simulink model "HEMS_1GDL_DISCRETIZADO"  (R2026b)
settings: Solver=VariableStepAuto  StopTime=5  MaxStep=1e-4
undefined symbols (not defined in the file): airgap_bp, airgap_zero_current, current_bp, Fz_table, g0, I_ff, I_initial, I_max, Kd_cur, Kd_pos, Ki_cur, Ki_pos, Kp_cur, Kp_pos, L_coil, m, N_pos, R_coil, Ts_cur, Ts_pos, v_initial, V_max, z_initial
libraries: slpidlib x2
settings Model: Creator=34666  LastModifiedBy=34666

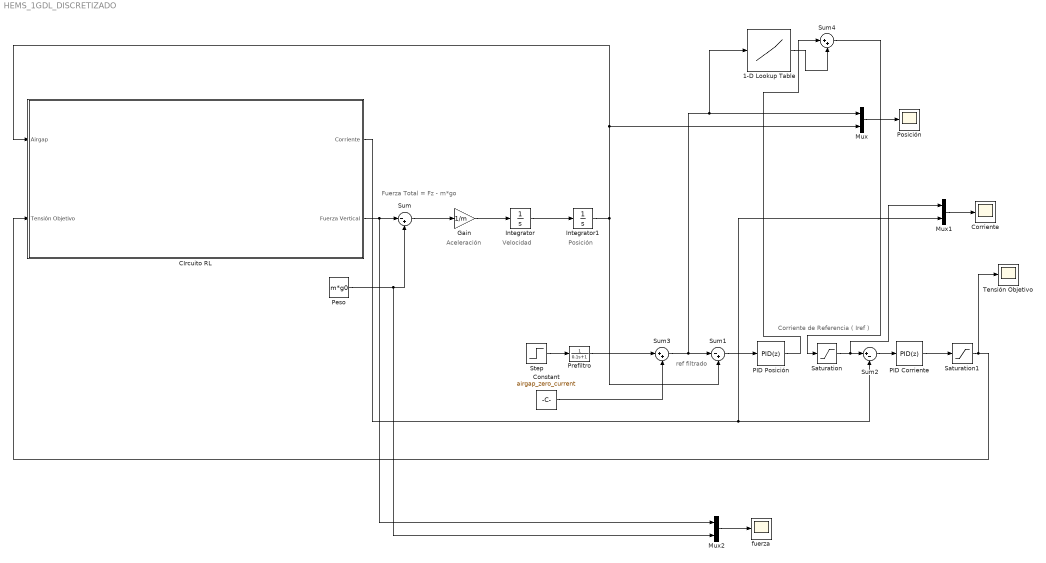
== system HEMS_1GDL_DISCRETIZADO ==
  note: ref filtrado
  note: Corriente de Referencia ( Iref )
  note: Aceleración
  note: Fuerza Total = Fz - m*go
  note: Velocidad
  note: Posición
  1-D Lookup Table : Lookup_n-D  NumberOfTableDimensions=1  BreakpointsForDimension1=airgap_bp  Table=I_ff  ExtrapMethod=Clip  InternalRulePriority=Speed  RndMeth=Simplest
  CIrcuito RL : Subsystem
  Constant : Constant  Value=airgap_zero_current
  Corriente : Scope
      settings: ActiveDisplayYMinimum=-30.569144829909195  ActiveDisplayYMaximum=22.357809311337615  DataLoggingVariableName=ScopeData2
  Gain : Gain  Gain=1/m
  Integrator : Integrator  InitialCondition=v_initial
  Integrator1 : Integrator  InitialCondition=z_initial
  Mux : Mux  Inputs=2
  Mux1 : Mux  Inputs=2
  Mux2 : Mux  Inputs=2
  PID Corriente : slpidlib/PID Controller  Controller=PID  Form=Parallel  TimeDomain=Discrete-time  UseExternalTs=off  SampleTime=Ts_cur  IntegratorMethod=Forward Euler  FilterMethod=Forward Euler  ControllerParametersSource=internal  P=Kp_cur  I=Ki_cur  UseKiTs=off  D=Kd_cur  UseExternalDerivativeSource=off  N=100  UseFilter=on  TunerSelectOption=Transfer Function Based (PID Tuner App)  InitialConditionSource=internal  InitialConditionForIntegrator=0  InitialConditionForFilter=0  DifferentiatorICPrevScaledInput=0  ExternalReset=none  TrackingMode=off  Kt=1  LimitOutput=on  SatLimitsSource=internal  UpperSaturationLimit=V_max  LowerSaturationLimit=-V_max  LinearizeAsGain=on  AntiWindupMode=back-calculation  Kb=1  LimitIntegrator=off  UpperIntegratorSaturationLimit=inf  LowerIntegratorSaturationLimit=-inf  POutMin=[]  POutMax=[]  IOutMin=[]  IOutMax=[]  DOutMin=[]  DOutMax=[]  NOutMin=[]  NOutMax=[]  SumOutMin=[]  SumOutMax=[]  SaturationOutMin=[]  SaturationOutMax=[]  PParamMin=[]  PParamMax=[]  IParamMin=[]  IParamMax=[]  DParamMin=[]  DParamMax=[]  NParamMin=[]  NParamMax=[]  KbParamMin=[]  KbParamMax=[]  KtParamMin=[]  KtParamMax=[]  KbOutMin=[]  KbOutMax=[]  KtOutMin=[]  KtOutMax=[]  IntegratorOutMin=[]  IntegratorOutMax=[]  FilterOutMin=[]  FilterOutMax=[]  SumI1OutMin=[]  SumI1OutMax=[]  SumI2OutMin=[]  SumI2OutMax=[]  SumI3OutMin=[]  SumI3OutMax=[]  SumI4OutMin=[]  SumI4OutMax=[]  SumDOutMin=[]  SumDOutMax=[]  DifferentiatorOutMin=[]  DifferentiatorOutMax=[]  FilterDiffOutCoefMin=[]  FilterDiffOutCoefMax=[]  ReciprocalOutMin=[]  ReciprocalOutMax=[]  SumDenOutMin=[]  SumDenOutMax=[]  SumNumOutMin=[]  SumNumOutMax=[]  DivideOutMin=[]  DivideOutMax=[]  UdiffTsProdOutMin=[]  UdiffTsProdOutMax=[]  NTsProdOutMin=[]  NTsProdOutMax=[]  UintegralTsProdOutMin=[]  UintegralTsProdOutMax=[]  UngainTsProdOutMin=[]  UngainTsProdOutMax=[]  ClampingZeroOutDataTypeStr=Inherit: Inherit via back propagation  ClampingZeroOutMin=[]  ClampingZeroOutMax=[]  FilterDenConstantOutDataTypeStr=Inherit: Inherit via back propagation  FilterDenConstantOutMin=[]  FilterDenConstantOutMax=[]  PCopyOutDataTypeStr=Inherit: Inherit via back propagation  PCopyOutMin=[]  PCopyOutMax=[]  NCopyOutDataTypeStr=Inherit: Inherit via back propagation  NCopyOutMin=[]  NCopyOutMax=[]  IntegratorContinuousStateAttributes=''  IntegratorStateMustResolveToSignalObject=off  IntegratorRTWStateStorageClass=Auto  FilterContinuousStateAttributes=''  FilterStateMustResolveToSignalObject=off  FilterRTWStateStorageClass=Auto  ParallelPVariant=InternalParameters  IdealPVariant=Disabled  IVariant=InternalParameters  DVariant=InternalParameters  IntegratorVariant=Discrete  SatVariant=Enabled  AWVariant=BackCalculation  PCopyVariant=Disabled  TRVariant=Disabled  FdbkBlocksVariant=Forward  IdealPFdbkVariant=Disabled  SatFdbkVariant=Disabled  DerivativeFilterVariant=ForwardEulerFilter  NVariant=InternalParameters  NCopyVariant=Disabled  FilterICVariant=InternalICsFilter  IntegratorICVariant=InternalICs  ExternalResetVariant=Disabled  TRSumVariant=Passthrough  SumFdbkVariant=Disabled  SumVariant=Sum_PID  TsampFilterVariant=InternalTs  TsampNgainVariant=Passthrough  TsampIntegralVariant=Disabled_SignalSpec  ExternalSaturationOutDataTypeStr=Inherit: Same as second input  DerivativeSourceVariant=ErrorSignal  PreIntVariant=InternalPreInt
  PID Posición : slpidlib/PID Controller  Controller=PID  Form=Parallel  TimeDomain=Discrete-time  UseExternalTs=off  SampleTime=Ts_pos  IntegratorMethod=Forward Euler  FilterMethod=Forward Euler  ControllerParametersSource=internal  P=Kp_pos  I=Ki_pos  UseKiTs=off  D=Kd_pos  UseExternalDerivativeSource=off  N=N_pos  UseFilter=on  TunerSelectOption=Transfer Function Based (PID Tuner App)  InitialConditionSource=internal  InitialConditionForIntegrator=0  InitialConditionForFilter=0  DifferentiatorICPrevScaledInput=0  ExternalReset=none  TrackingMode=off  Kt=1  LimitOutput=on  SatLimitsSource=internal  UpperSaturationLimit=I_max  LowerSaturationLimit=-I_max  LinearizeAsGain=on  AntiWindupMode=back-calculation  Kb=1  LimitIntegrator=off  UpperIntegratorSaturationLimit=inf  LowerIntegratorSaturationLimit=-inf  POutMin=[]  POutMax=[]  IOutMin=[]  IOutMax=[]  DOutMin=[]  DOutMax=[]  NOutMin=[]  NOutMax=[]  SumOutMin=[]  SumOutMax=[]  SaturationOutMin=[]  SaturationOutMax=[]  PParamMin=[]  PParamMax=[]  IParamMin=[]  IParamMax=[]  DParamMin=[]  DParamMax=[]  NParamMin=[]  NParamMax=[]  KbParamMin=[]  KbParamMax=[]  KtParamMin=[]  KtParamMax=[]  KbOutMin=[]  KbOutMax=[]  KtOutMin=[]  KtOutMax=[]  IntegratorOutMin=[]  IntegratorOutMax=[]  FilterOutMin=[]  FilterOutMax=[]  SumI1OutMin=[]  SumI1OutMax=[]  SumI2OutMin=[]  SumI2OutMax=[]  SumI3OutMin=[]  SumI3OutMax=[]  SumI4OutMin=[]  SumI4OutMax=[]  SumDOutMin=[]  SumDOutMax=[]  DifferentiatorOutMin=[]  DifferentiatorOutMax=[]  FilterDiffOutCoefMin=[]  FilterDiffOutCoefMax=[]  ReciprocalOutMin=[]  ReciprocalOutMax=[]  SumDenOutMin=[]  SumDenOutMax=[]  SumNumOutMin=[]  SumNumOutMax=[]  DivideOutMin=[]  DivideOutMax=[]  UdiffTsProdOutMin=[]  UdiffTsProdOutMax=[]  NTsProdOutMin=[]  NTsProdOutMax=[]  UintegralTsProdOutMin=[]  UintegralTsProdOutMax=[]  UngainTsProdOutMin=[]  UngainTsProdOutMax=[]  ClampingZeroOutDataTypeStr=Inherit: Inherit via back propagation  ClampingZeroOutMin=[]  ClampingZeroOutMax=[]  FilterDenConstantOutDataTypeStr=Inherit: Inherit via back propagation  FilterDenConstantOutMin=[]  FilterDenConstantOutMax=[]  PCopyOutDataTypeStr=Inherit: Inherit via back propagation  PCopyOutMin=[]  PCopyOutMax=[]  NCopyOutDataTypeStr=Inherit: Inherit via back propagation  NCopyOutMin=[]  NCopyOutMax=[]  IntegratorContinuousStateAttributes=''  IntegratorStateMustResolveToSignalObject=off  IntegratorRTWStateStorageClass=Auto  FilterContinuousStateAttributes=''  FilterStateMustResolveToSignalObject=off  FilterRTWStateStorageClass=Auto  ParallelPVariant=InternalParameters  IdealPVariant=Disabled  IVariant=InternalParameters  DVariant=InternalParameters  IntegratorVariant=Discrete  SatVariant=Enabled  AWVariant=BackCalculation  PCopyVariant=Disabled  TRVariant=Disabled  FdbkBlocksVariant=Forward  IdealPFdbkVariant=Disabled  SatFdbkVariant=Disabled  DerivativeFilterVariant=ForwardEulerFilter  NVariant=InternalParameters  NCopyVariant=Disabled  FilterICVariant=InternalICsFilter  IntegratorICVariant=InternalICs  ExternalResetVariant=Disabled  TRSumVariant=Passthrough  SumFdbkVariant=Disabled  SumVariant=Sum_PID  TsampFilterVariant=InternalTs  TsampNgainVariant=Passthrough  TsampIntegralVariant=Disabled_SignalSpec  ExternalSaturationOutDataTypeStr=Inherit: Same as second input  DerivativeSourceVariant=ErrorSignal  PreIntVariant=InternalPreInt
  Peso : Constant  Value=m*g0
  Posición : Scope
      settings: ActiveDisplayYMinimum=0.010559924308115764  ActiveDisplayYMaximum=0.02352298260570624
  Prefiltro : TransferFcn  Denominator=[0.1 1]
  Saturation : Saturate  UpperLimit=I_max  LowerLimit=-I_max
  Saturation1 : Saturate  UpperLimit=V_max  LowerLimit=-V_max
  Step : Step  FinalValue=0.018-airgap_zero_current  SampleTime=0
  Sum : Sum  Inputs=|-+
  Sum1 : Sum  Inputs=|-+
  Sum2 : Sum  Inputs=|+-
  Sum3 : Sum  Inputs=|++
  Sum4 : Sum  Inputs=|++
  Tensión Objetivo : Scope
      settings: ActiveDisplayYMinimum=2.092085175210403  ActiveDisplayYMaximum=3.7936508221223049
  fuerza : Scope
      settings: ActiveDisplayYMinimum=349.8545191819162  ActiveDisplayYMaximum=731.51535099662465  DataLoggingVariableName=ScopeData3
  wires:
  CIrcuito RL/2(Fuerza Vertical) -> Mux2/1, Sum/1
  Peso/1 -> Mux2/2, Sum/2
  Sum/1 -> Gain/1
  Gain/1 -> Integrator/1
  Integrator/1 -> Integrator1/1
  Integrator1/1 -> Sum1/2, Mux/2, CIrcuito RL/1(Airgap)
  Sum1/1 -> PID Posición/1
  Saturation/1 -> Mux1/1, Sum2/1
  CIrcuito RL/1("Corriente ") -> Sum2/2, Mux1/2
  Sum2/1 -> PID Corriente/1
  PID Corriente/1 -> Saturation1/1
  Saturation1/1 -> Tensión Objetivo/1, CIrcuito RL/2("Tensión Objetivo ")
  Mux/1 -> Posición/1
  Mux1/1 -> Corriente/1
  Mux2/1 -> fuerza/1
  Step/1 -> Prefiltro/1
  Prefiltro/1 -> Sum3/1
  Constant/1 -> Sum3/2
  Sum3/1 -> 1-D Lookup Table/1, Mux/1, Sum1/1
  PID Posición/1 -> Sum4/1
  1-D Lookup Table/1 -> Sum4/2
  Sum4/1 -> Saturation/1

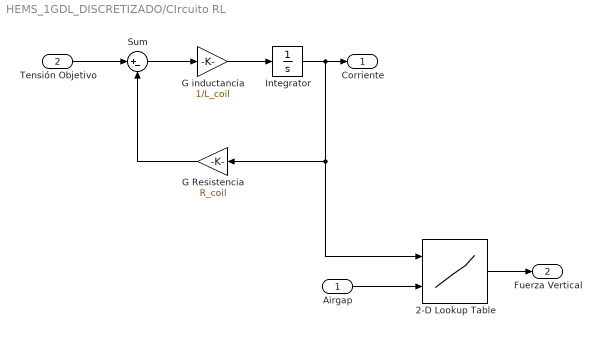
== system HEMS_1GDL_DISCRETIZADO/CIrcuito RL ==
  Airgap : Inport
  "Tensión Objetivo " : Inport  Port=2
  2-D Lookup Table : Lookup_n-D  BreakpointsForDimension1=current_bp  BreakpointsForDimension2=airgap_bp  Table=Fz_table  ExtrapMethod=Clip  InternalRulePriority=Speed  RndMeth=Simplest
      settings: InputPortMap=u0,u1
  G Resistencia : Gain  Gain=R_coil
  G inductancia : Gain  Gain=1/L_coil
  Integrator : Integrator  InitialCondition=I_initial
  Sum : Sum  Inputs=|+-
  "Corriente " : Outport
  Fuerza Vertical : Outport  Port=2
  wires:
  "Tensión Objetivo "/1 -> Sum/1
  Sum/1 -> G inductancia/1
  G inductancia/1 -> Integrator/1
  Integrator/1 -> G Resistencia/1, 2-D Lookup Table/1, "Corriente "/1
  G Resistencia/1 -> Sum/2
  Airgap/1 -> 2-D Lookup Table/2
  2-D Lookup Table/1 -> Fuerza Vertical/1
